simulink library "lindiPlane_lib"  (R2023b)
settings: Solver=VariableStepAuto  StartTime=0.0  StopTime=10.0  RelTol=1e-3
undefined symbols (not defined in the file or in its folder): DiscIntNeverNeededParam, lindi, lindi_notune
libraries: filters_lib x28, $bdroot x20, simulink x12, ca_lib x2, axes_transformation_lib x1, unit_conversions_lib x1, wpnav_lib x1
(part 1 of 2)
settings Model: Creator=Ybeyer  LastModifiedBy=yannic
settings SolverCC: AlgebraicLoopSolver=TrustRegion
settings DataIOCC: ReturnWorkspaceOutputs=off
settings DebuggingCC: UnconnectedInputMsg=warning  UnconnectedOutputMsg=warning  UnconnectedLineMsg=warning  ArithmeticOperatorsInVariantConditions=warning
settings ModelReferenceCC: EnableRefExpFcnMdlSchedulingChecks=on
settings SFSimCC: SimUseLocalCustomCode=off  CustomCodeUndefinedFunction=UseInterfaceOnly
settings RTWCC: RTWUseLocalCustomCode=off
settings CodeAppCC: StateflowObjectComments=on

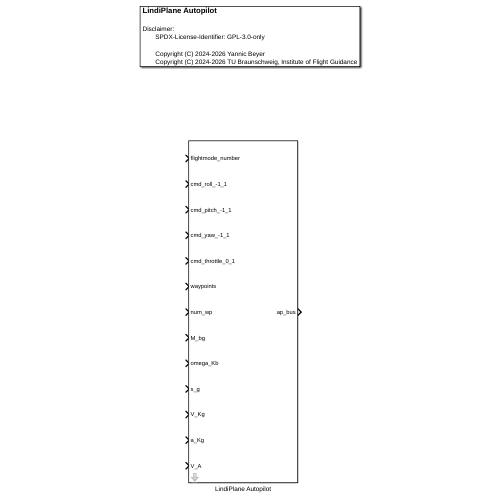
[thumbnail: Simulink's stored preview of the top-level diagram]
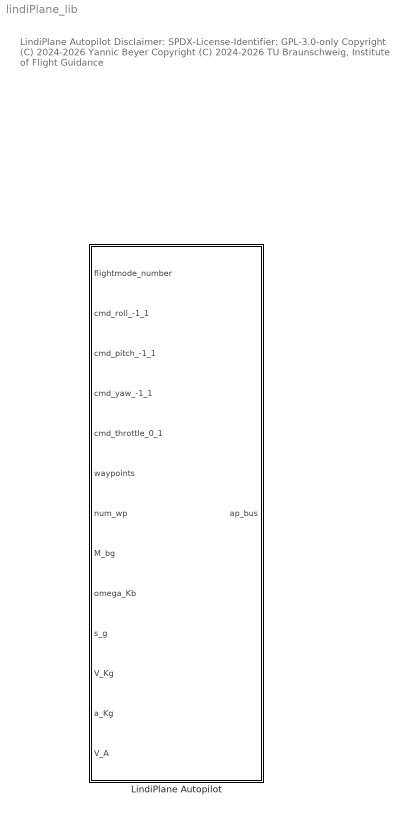
== system lindiPlane_lib ==
  note: LindiPlane Autopilot
      |
      | Disclaimer:
      | SPDX-License-Identifier: GPL-3.0-only
      |
      | Copyright (C) 2024-2026 Yannic Beyer
      | Copyright (C) 2024-2026 TU Braunschweig, Institute of Flight Guidance
  LindiPlane Autopilot : Subsystem  mask{ap=lindi, ap_notune=lindi_notune, is_enable_checked=off, states_when_enabling=reset, is_cmd_wrbm_n=off}
      mask prompts: ap "LindiPlane parameters struct, see lindiPlaneAutoCreate"; ap_notune "LindiPlane non-tunable parameters struct"; is_enable_checked "Activate "Enabled Subsystem""; states_when_enabling "States when enabling:"; is_cmd_wrbm_n "Enable WRBM load factor command"
      mask init:
      | % blockInitToggleEnable(is_enable_checked,states_when_enabling);
      | cntrlBlockInit(is_enable_checked,states_when_enabling);
      | blockInitToggleInport('cmd_WRBM_n', is_cmd_wrbm_n);
      mask Help: web('https://github.com/iff-gsc/LADAC/blob/main/control/autopilots/LindiPlane/README.md','-browser')
      mask TypeOptions states_when_enabling: held | reset
      mask DialogControl DescGroupVar Prompt: LindiPlane Autopilot
      mask DialogControl DescTextVar Prompt: The documentation of this block can be found here
      mask DialogControl Control2 Prompt: README
      mask DialogControl Control2 Callback: web('https://github.com/iff-gsc/LADAC/blob/main/control/autopilots/LindiPlane/README.md','-browser')

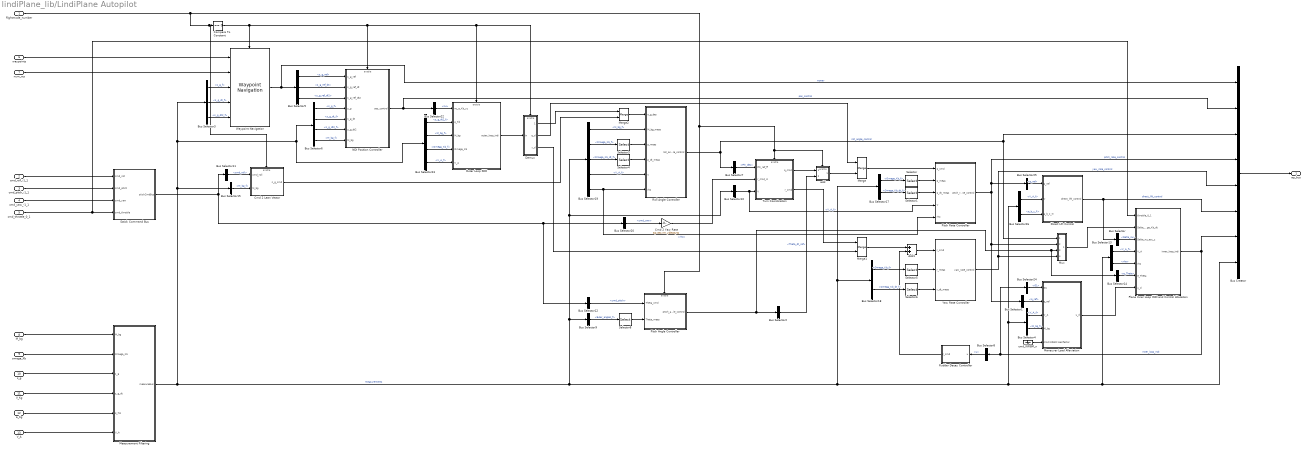
== system lindiPlane_lib/LindiPlane Autopilot ==
  flightmode_number : Inport
  cmd_roll_-1_1 : Inport  Port=2
  cmd_pitch_-1_1 : Inport  Port=3
  cmd_yaw_-1_1 : Inport  Port=4
  cmd_throttle_0_1 : Inport  Port=5
  waypoints : Inport  Port=6
  num_wp : Inport  Port=7
  M_bg : Inport  Port=8
  omega_Kb : Inport  Port=9
  s_g : Inport  Port=10
  V_Kg : Inport  Port=11
  a_Kg : Inport  Port=12
  V_A : Inport  Port=13
  Add1 : Sum
  Bus Creator : BusCreator  Inputs=8
  Bus Selector : BusSelector  OutputSignals=Delta_nu
  Bus Selector1 : BusSelector  OutputSignals=reference.q_ref
  Bus Selector10 : BusSelector  OutputSignals=V_A_f
  Bus Selector11 : BusSelector  OutputSignals=cmd_roll
  Bus Selector12 : BusSelector  OutputSignals=cmd_pitch
  Bus Selector13 : BusSelector  OutputSignals=V_A_f,rho
  Bus Selector14 : BusSelector  OutputSignals=e_Theta
  Bus Selector15 : BusSelector  OutputSignals=M_bg_f
  Bus Selector17 : BusSelector  OutputSignals=Omega_Kb_f,Omega_Kb_dt_f
  Bus Selector18 : BusSelector  OutputSignals=Omega_Kb_f,Omega_Kb_dt_f
  Bus Selector19 : BusSelector  OutputSignals=M_bg_f,Omega_Kb_f,Omega_Kb_dt_f,V_A_f,rho
  Bus Selector2 : BusSelector  OutputSignals=Theta_dt_ref
  Bus Selector20 : BusSelector  OutputSignals=cmd_yaw
  Bus Selector22 : BusSelector  OutputSignals=pseudo_control.nu
  Bus Selector23 : BusSelector  OutputSignals=s_g_dt2_f,M_bg_f,Omega_Kb_f,V_A_f
  Bus Selector24 : BusSelector  OutputSignals=G1
  Bus Selector25 : BusSelector  OutputSignals=reference.q_ref
  Bus Selector26 : BusSelector  OutputSignals=V_A_f,a_b_z_F
  Bus Selector3 : BusSelector  OutputSignals=s_g_f,s_g_dt_f,s_g_dt2_f
  Bus Selector4 : BusSelector  OutputSignals=V_A_f,M_bg_f
  Bus Selector5 : BusSelector  OutputSignals=ref_smooth.s_g_ref,ref_smooth.s_g_ref_dt,ref_smooth.s_g_ref_dt2
  Bus Selector6 : BusSelector  OutputSignals=s_g_f,s_g_dt_f,s_g_dt2_f,M_bg_f
  Bus Selector7 : BusSelector  OutputSignals=reference.Phi_des
  Bus Selector8 : BusSelector  OutputSignals=u
  Bus Selector9 : BusSelector  OutputSignals=Euler_angles_f
  Cmd 2 Lean Vector : Subsystem
  Cmd 2 Yaw Rate : Gain  Gain=ap.atc.rm.ydecaytc
  Compare To Constant : simulink/Logic and Bit Operations/Compare To Constant  relop===  const=0  OutDataTypeStr=boolean
  Demux : Subsystem
  Direct Lift Control : Subsystem
  Maneuver Load Alleviation : Subsystem
  Measurement Filtering : Subsystem
  Merge : Merge
  Merge1 : Merge
  Merge2 : Merge
  Mux : Subsystem
  NDI Position Controller : Subsystem
  Outer Loop INDI : Subsystem
  Pitch Angle Controller : Subsystem
  Pitch Rate Controller : Subsystem
  Plane Inner Loop INDI and Control Allocation : Subsystem
  Roll Angle Controller : Subsystem
  Rudder Decay Controller : Subsystem
  Selector : Selector  InputPortWidth=3  IndexOptions=Index vector (dialog)  Indices=2  OutputSizes=1
  Selector1 : Selector  InputPortWidth=3  IndexOptions=Index vector (dialog)  Indices=2  OutputSizes=1
  Selector3 : Selector  InputPortWidth=3  IndexOptions=Index vector (dialog)  Indices=1  OutputSizes=1
  Selector4 : Selector  InputPortWidth=3  IndexOptions=Index vector (dialog)  Indices=1  OutputSizes=1
  Selector5 : Selector  InputPortWidth=3  IndexOptions=Index vector (dialog)  Indices=3  OutputSizes=1
  Selector6 : Selector  InputPortWidth=3  IndexOptions=Index vector (dialog)  Indices=3  OutputSizes=1
  Selector8 : Selector  InputPortWidth=3  IndexOptions=Index vector (dialog)  Indices=2  OutputSizes=1
  Sstick Command Bus : Subsystem
  Turn Coordination : Subsystem
  Waypoint Navigation : wpnav_lib/Waypoint Navigation  wpnav=ap.wpnav  T_inner_loop=2/ap.atc.rm.rfreq + 2/(ap.servo.boost*ap.servo.omega) + 2/ap.sflt.omega  is_enable_checked=on  states_when_enabling=held  mask_expr_handling_config=passthrough (tunable)
      settings: SourceProductName=LADAC
  Yaw Rate Controller : Subsystem
  add : Subsystem
  cmd_WRBM_n : Ground
  ap_bus : Outport  VectorParamsAs1DForOutWhenUnconnected=off
  wires:
  Bus Selector15/1 -> Cmd 2 Lean Vector/2(M_bg)  "<M_bg_f>"
  cmd_WRBM_n/1 -> Maneuver Load Alleviation/5(cmd WRBM load factor)
  Bus Selector5/3 -> NDI Position Controller/3(s_g_ref_dt2)  "<s_g_ref_dt2>"
  Bus Selector5/2 -> NDI Position Controller/2(s_g_ref_dt)  "<s_g_ref_dt>"
  Bus Selector5/1 -> NDI Position Controller/1(s_g_ref)  "<s_g_ref>"
  Bus Selector14/1 -> Plane Inner Loop INDI and Control Allocation/6(e_Theta)  "<e_Theta>"
  Mux/1(Om) -> Plane Inner Loop INDI and Control Allocation/2(Delta_nu_Omega_Kb_dt)
  Bus Selector/1 -> Plane Inner Loop INDI and Control Allocation/3(Delta_nu_acc_z)  "<Delta_nu>"
  Direct Lift Control/1(direct_lift_control) -> Bus Creator/6, Bus Selector/1  "direct_lift_control"
  Bus Selector26/2 -> Direct Lift Control/3(a_b_z_N)  "<a_b_z_F>"
  Bus Selector26/1 -> Direct Lift Control/2(V)  "<V_A_f>"
  Bus Selector25/1 -> Direct Lift Control/1(q_ref)  "<q_ref>"
  waypoints/1 -> Waypoint Navigation/1
  Bus Selector19/5 -> Roll Angle Controller/6(rho), Pitch Rate Controller/5(rho)  "<rho>"
  Bus Selector19/4 -> Roll Angle Controller/5(V)  "<V_A_f>"
  Bus Selector13/2 -> Plane Inner Loop INDI and Control Allocation/5(rho)  "<rho>"
  num_wp/1 -> Waypoint Navigation/2
  NDI Position Controller/1(pos_control) -> Bus Creator/2, Bus Selector22/1  "pos_control"
  Bus Creator/1 -> ap_bus/1
  M_bg/1 -> Measurement Filtering/1(M_bg)
  omega_Kb/1 -> Measurement Filtering/2(Omega_Kb)
  s_g/1 -> Measurement Filtering/3(s_g)
  V_Kg/1 -> Measurement Filtering/4(s_g_dt)
  a_Kg/1 -> Measurement Filtering/5(a_Kg)
  V_A/1 -> Measurement Filtering/6(V_A)
  Bus Selector12/1 -> Pitch Angle Controller/1(Theta_cmd)  "<cmd_pitch>"
  Bus Selector6/2 -> NDI Position Controller/5(s_g_dt)  "<s_g_dt_f>"
  Measurement Filtering/1(measureBus) -> Bus Selector19/1, Bus Selector10/1, Bus Selector9/1, Bus Selector17/1, Bus Selector18/1, Bus Creator/8, Bus Selector13/1, Bus Selector4/1, Bus Selector26/1, Bus Selector23/1, Bus Selector6/1, Bus Selector3/1, Bus Selector15/1  "measurements"
  Bus Selector8/1 -> Rudder Decay Controller/1(u)  "<u>"
  Yaw Rate Controller/1(yaw_rate_control) -> Mux/4(yaw), Bus Creator/5  "yaw_rate_control"
  cmd_yaw_-1_1/1 -> Sstick Command Bus/3(cmd_yaw)
  Bus Selector13/1 -> Plane Inner Loop INDI and Control Allocation/4(V_A)  "<V_A_f>"
  flightmode_number/1 -> Cmd 2 Lean Vector/Enable, Compare To Constant/1, add/Enable, Turn Coordination/Enable, Pitch Angle Controller/Enable
  Bus Selector18/2 -> Selector6/1  "<Omega_Kb_dt_f>"
  Selector4/1 -> Roll Angle Controller/4(p_dt_meas)
  Cmd 2 Lean Vector/1(n_g_cmd) -> Merge2/2
  Bus Selector3/2 -> Waypoint Navigation/4  "<s_g_dt_f>"
  Bus Selector17/1 -> Selector/1  "<Omega_Kb_f>"
  Selector6/1 -> Yaw Rate Controller/3(r_dt_meas)
  Selector5/1 -> Yaw Rate Controller/2(r_meas)
  Roll Angle Controller/1(roll_angle_control) -> Bus Creator/3, Mux/1(rll), Bus Selector7/1  "roll_angle_control"
  Merge1/1 -> Add1/1
  Selector8/1 -> Pitch Angle Controller/2(Theta_meas)
  cmd_throttle_0_1/1 -> Plane Inner Loop INDI and Control Allocation/1(throttle_0_1), Sstick Command Bus/4(cmd_throttle)
  Pitch Rate Controller/1(pitch_rate_control) -> Mux/2(ptch), Bus Selector1/1, Bus Selector25/1, Bus Creator/4  "pitch_rate_control"
  Bus Selector6/3 -> NDI Position Controller/6(s_g_dt2)  "<s_g_dt2_f>"
  Turn Coordination/2(r_cmd) -> Merge1/1
  Selector3/1 -> Roll Angle Controller/3(p_meas)
  Waypoint Navigation/1 -> Bus Selector5/1, Bus Creator/1  "wpnav"
  Bus Selector10/1 -> Turn Coordination/3(V), Pitch Rate Controller/4(V)  "<V_A_f>"
  Selector1/1 -> Pitch Rate Controller/3(q_dt_meas)
  cmd_pitch_-1_1/1 -> Sstick Command Bus/2(cmd_pitch)
  Selector/1 -> Pitch Rate Controller/2(q_meas)
  Bus Selector19/2 -> Selector3/1  "<Omega_Kb_f>"
  Compare To Constant/1 -> Waypoint Navigation/Enable, Demux/Enable, Outer Loop INDI/Enable, NDI Position Controller/Enable
  Cmd 2 Yaw Rate/1 -> Turn Coordination/2(r_cmd_in)
  Bus Selector3/1 -> Waypoint Navigation/3  "<s_g_f>"
  Sstick Command Bus/1(stickCmdBus) -> Bus Selector11/1, Bus Selector20/1, Bus Selector12/1
  Bus Selector9/1 -> Selector8/1  "<Euler_angles_f>"
  Rudder Decay Controller/1(r_cmd) -> Add1/2
  Bus Selector19/3 -> Selector4/1  "<Omega_Kb_dt_f>"
  Bus Selector17/2 -> Selector1/1  "<Omega_Kb_dt_f>"
  Bus Selector11/1 -> Cmd 2 Lean Vector/1(cmd_roll)  "<cmd_roll>"
  Bus Selector2/1 -> add/2(In2)  "<Theta_dt_ref>"
  cmd_roll_-1_1/1 -> Sstick Command Bus/1(cmd_roll)
  Bus Selector19/1 -> Roll Angle Controller/2(M_bg_meas)  "<M_bg_f>"
  Bus Selector6/1 -> NDI Position Controller/4(s_g)  "<s_g_f>"
  Plane Inner Loop INDI and Control Allocation/1(inner_loop_indi) -> Bus Creator/7, Bus Selector8/1, Bus Selector24/1  "inner_loop_indi"
  Bus Selector6/4 -> NDI Position Controller/7(M_bg)  "<M_bg_f>"
  Bus Selector18/1 -> Selector5/1  "<Omega_Kb_f>"
  Add1/1 -> Yaw Rate Controller/1(r_cmd)
  Merge2/1 -> Roll Angle Controller/1(n_g_des)
  Bus Selector20/1 -> Cmd 2 Yaw Rate/1  "<cmd_yaw>"
  Bus Selector3/3 -> Waypoint Navigation/5  "<s_g_dt2_f>"
  Merge/1 -> Pitch Rate Controller/1(q_cmd)
  Turn Coordination/1(q_cmd) -> add/1(In1)
  add/1(Out1) -> Merge/2
  Pitch Angle Controller/1(pitch_angle_control) -> Bus Selector2/1, Mux/3(ptch2), Bus Selector14/1
  Outer Loop INDI/1(outer_loop_indi) -> Demux/1(In)
  Demux/2(q_d) -> Merge/1
  Demux/3(r_d) -> Merge1/2
  Demux/1(n_g_d) -> Merge2/1
  Bus Selector7/1 -> Turn Coordination/1(Phi_ref_ff)  "<Phi_des>"
  Bus Selector22/1 -> Outer Loop INDI/1(nu_a_Kb_yz)  "<nu>"
  Bus Selector23/4 -> Outer Loop INDI/5(V_A)  "<V_A_f>"
  Bus Selector23/3 -> Outer Loop INDI/4(Omega_Kb)  "<Omega_Kb_f>"
  Bus Selector23/2 -> Outer Loop INDI/3(M_bg)  "<M_bg_f>"
  Bus Selector23/1 -> Outer Loop INDI/2(a_Kb)  "<s_g_dt2_f>"
  Bus Selector1/1 -> Maneuver Load Alleviation/2(q_ref)  "<q_ref>"
  Bus Selector4/1 -> Maneuver Load Alleviation/3(V_A)  "<V_A_f>"
  Bus Selector4/2 -> Maneuver Load Alleviation/4(M_bg)  "<M_bg_f>"
  Bus Selector24/1 -> Maneuver Load Alleviation/1(G1)  "<G1>"
  Maneuver Load Alleviation/1(u_d) -> Plane Inner Loop INDI and Control Allocation/7(u_d)

== system lindiPlane_lib/LindiPlane Autopilot/Cmd 2 Lean Vector ==
  cmd_roll : Inport
  M_bg : Inport  Port=2
  Enable : EnablePort
  Cmd Roll 2 n_g_cmd : MATLAB Function  TreatAsAtomicUnit=on
  Gain : Gain  Gain=ap.atc.rm.rangmax*pi/180
  n_g_cmd : Outport  VectorParamsAs1DForOutWhenUnconnected=off
  wires:
  M_bg/1 -> Cmd Roll 2 n_g_cmd/2(M_bg)
  Cmd Roll 2 n_g_cmd/1(n_g_cmd) -> n_g_cmd/1
  Gain/1 -> Cmd Roll 2 n_g_cmd/1(Phi_cmd)
  cmd_roll/1 -> Gain/1

== system lindiPlane_lib/LindiPlane Autopilot/Demux ==
  In : Inport
  Enable : EnablePort
  Bus Selector24 : BusSelector  OutputSignals=n_g_des,q_des,r_des
  n_g_d : Outport  VectorParamsAs1DForOutWhenUnconnected=off
  q_d : Outport  Port=2  VectorParamsAs1DForOutWhenUnconnected=off
  r_d : Outport  Port=3  VectorParamsAs1DForOutWhenUnconnected=off
  wires:
  Bus Selector24/1 -> n_g_d/1  "<n_g_des>"
  In/1 -> Bus Selector24/1
  Bus Selector24/2 -> q_d/1  "<q_des>"
  Bus Selector24/3 -> r_d/1  "<r_des>"

== system lindiPlane_lib/LindiPlane Autopilot/Direct Lift Control ==
  q_ref : Inport
  V : Inport  Port=2
  a_b_z_N : Inport  Port=3
  Acc Filter : $bdroot/LindiPlane Autopilot/Measurement Filtering/Acc Filter  SystemSampleTime=-1  VariantActivationTime=update diagram  AllowFlexibleInterface=on  Latency=0  AutoFrameSizeCalculation=off
  Add : Sum  Inputs=|+-
  Bus Creator : BusCreator  Inputs=4
  Gain1 : Gain  Gain=-1
  Product : Product
  Scope : Scope  NumInputPorts=3
  direct_lift_control : Outport  VectorParamsAs1DForOutWhenUnconnected=off
  wires:
  Acc Filter/1 -> Scope/2, Bus Creator/2  "nu_f"
  Gain1/1 -> Scope/1, Bus Creator/1, Acc Filter/1, Add/1  "nu"
  a_b_z_N/1 -> Scope/3, Bus Creator/4, Add/2  "nu_meas"
  Add/1 -> Bus Creator/3  "Delta_nu"
  V/1 -> Product/2
  Product/1 -> Gain1/1
  Bus Creator/1 -> direct_lift_control/1
  q_ref/1 -> Product/1

== system lindiPlane_lib/LindiPlane Autopilot/Maneuver Load Alleviation ==
  G1 : Inport
  q_ref : Inport  Port=2
  V_A : Inport  Port=3
  M_bg : Inport  Port=4
  cmd WRBM load factor : Inport  Port=5
  Compare To Constant : simulink/Logic and Bit Operations/Compare To Constant  relop===  const=0  OutDataTypeStr=boolean
  Constant : Constant  Value=ap.mla.use
  Logical Operator : Logic  Operator=NOT  AllPortsSameDT=off  OutDataTypeStr=boolean
  Maneuver Load Alleviation : Subsystem  mask{ca_main=ap.ca, ca_mla=ap.mla.ca}
      mask prompts: ca_main "Control allocation struct (main)"; ca_mla "Control allocation struct (MLA)"
      mask DialogControl DescGroupVar Prompt: Maneuver Load Alleviation (MLA)
  Merge : Merge
  Subsystem : Subsystem
  u_d : Outport  VectorParamsAs1DForOutWhenUnconnected=off
  wires:
  cmd WRBM load factor/1 -> Maneuver Load Alleviation/5(cmd WRBM load factor)
  M_bg/1 -> Maneuver Load Alleviation/4(M_bg)
  G1/1 -> Maneuver Load Alleviation/1(G1)
  q_ref/1 -> Maneuver Load Alleviation/3(q_ref)
  V_A/1 -> Maneuver Load Alleviation/2(V_A)
  Compare To Constant/1 -> Logical Operator/1, Subsystem/Enable
  Subsystem/1(u_d) -> Merge/1
  Constant/1 -> Compare To Constant/1
  Maneuver Load Alleviation/1(u_d) -> Merge/2
  Merge/1 -> u_d/1
  Logical Operator/1 -> Maneuver Load Alleviation/Enable

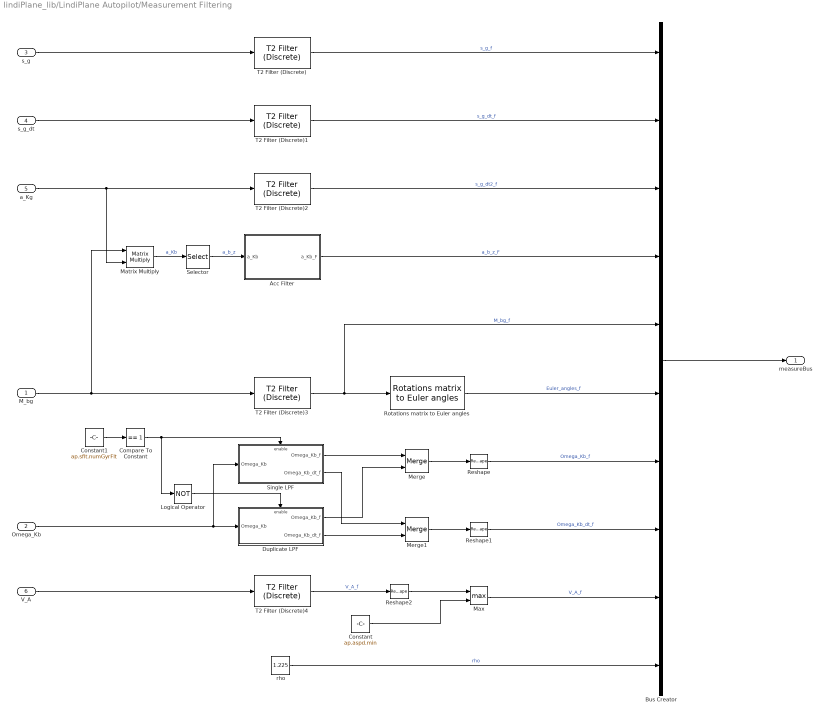
== system lindiPlane_lib/LindiPlane Autopilot/Measurement Filtering ==
  M_bg : Inport
  Omega_Kb : Inport  Port=2
  s_g : Inport  Port=3
  s_g_dt : Inport  Port=4
  a_Kg : Inport  Port=5
  V_A : Inport  Port=6
  Acc Filter : Subsystem
  Bus Creator : BusCreator  Inputs=10
  Compare To Constant : simulink/Logic and Bit Operations/Compare To Constant  relop===  const=1  OutDataTypeStr=boolean
  Constant : Constant  Value=ap.aspd.min
  Constant1 : Constant  Value=ap.sflt.numGyrFlt
  Duplicate LPF : Subsystem
  Logical Operator : Logic  Operator=NOT  AllPortsSameDT=off  OutDataTypeStr=boolean
  Matrix Multiply : Product  Multiplication=Matrix(*)
  Max : MinMax  Function=max  Inputs=2
  Merge : Merge
  Merge1 : Merge
  Reshape : Reshape  OutputDimensionality=Column vector (2-D)
  Reshape1 : Reshape  OutputDimensionality=Column vector (2-D)
  Reshape2 : Reshape
  Rotations matrix to Euler angles : axes_transformation_lib/Rotations matrix to Euler angles  SystemSampleTime=-1  VariantActivationTime=update diagram  AllowFlexibleInterface=on  Latency=0  AutoFrameSizeCalculation=off
      settings: SourceProductName=LADAC
  Selector : Selector  InputPortWidth=3  IndexOptions=Index vector (dialog)  Indices=3  OutputSizes=1
  Single LPF : Subsystem
  T2 Filter (Discrete){,1..3} (4 alike) : filters_lib/T2 Filter (Discrete)  omega_0=ap.sflt.omega  d=ap.sflt.d  Ts=ap_notune.ts  is_vel=false  is_acc=false  SimulateUsing=Code generation
      settings: SourceProductName=LADAC
  T2 Filter (Discrete)4 : filters_lib/T2 Filter (Discrete)  omega_0=2/ap.aspd.flttc  d=1  Ts=ap_notune.ts  is_vel=false  is_acc=false  SimulateUsing=Code generation
      settings: SourceProductName=LADAC
  rho : Constant  Value=1.225
  measureBus : Outport  VectorParamsAs1DForOutWhenUnconnected=off
  wires:
  Reshape2/1 -> Max/1
  Acc Filter/1(a_Kb_F) -> Bus Creator/4  "a_b_z_F"
  Selector/1 -> Acc Filter/1(a_Kb)  "a_b_z"
  Matrix Multiply/1 -> Selector/1  "a_Kb"
  M_bg/1 -> Matrix Multiply/1, T2 Filter (Discrete)3/1
  a_Kg/1 -> Matrix Multiply/2, T2 Filter (Discrete)2/1
  Logical Operator/1 -> Duplicate LPF/Enable
  Compare To Constant/1 -> Single LPF/Enable, Logical Operator/1
  Duplicate LPF/2(Omega_Kb_dt_f) -> Merge1/2
  Single LPF/2(Omega_Kb_dt_f) -> Merge1/1
  Duplicate LPF/1(Omega_Kb_f) -> Merge/2
  Single LPF/1(Omega_Kb_f) -> Merge/1
  Omega_Kb/1 -> Duplicate LPF/1(Omega_Kb), Single LPF/1(Omega_Kb)
  Constant1/1 -> Compare To Constant/1
  Reshape1/1 -> Bus Creator/8  "Omega_Kb_dt_f"
  Reshape/1 -> Bus Creator/7  "Omega_Kb_f"
  Merge/1 -> Reshape/1
  rho/1 -> Bus Creator/10  "rho"
  Constant/1 -> Max/2
  T2 Filter (Discrete)4/1 -> Reshape2/1  "V_A_f"
  Max/1 -> Bus Creator/9  "V_A_f"
  T2 Filter (Discrete)1/1 -> Bus Creator/2  "s_g_dt_f"
  T2 Filter (Discrete)/1 -> Bus Creator/1  "s_g_f"
  Bus Creator/1 -> measureBus/1
  T2 Filter (Discrete)2/1 -> Bus Creator/3  "s_g_dt2_f"
  Merge1/1 -> Reshape1/1
  V_A/1 -> T2 Filter (Discrete)4/1
  s_g/1 -> T2 Filter (Discrete)/1
  Rotations matrix to Euler angles/1 -> Bus Creator/6  "Euler_angles_f"
  T2 Filter (Discrete)3/1 -> Rotations matrix to Euler angles/1, Bus Creator/5  "M_bg_f"
  s_g_dt/1 -> T2 Filter (Discrete)1/1

== system lindiPlane_lib/LindiPlane Autopilot/Mux ==
  rll : Inport
  ptch : Inport  Port=2
  ptch2 : Inport  Port=3
  yaw : Inport  Port=4
  Add : Sum
  Bus Selector14 : BusSelector  OutputSignals=pseudo_control.Delta_nu
  Bus Selector15 : BusSelector  OutputSignals=pseudo_control.Delta_nu
  Bus Selector16 : BusSelector  OutputSignals=pseudo_control.Delta_nu
  Bus Selector21 : BusSelector  OutputSignals=nu_q_dt_ptchcntrl
  Mux2 : Mux  Inputs=3
  Om : Outport  VectorParamsAs1DForOutWhenUnconnected=off
  wires:
  ptch/1 -> Bus Selector15/1
  Bus Selector21/1 -> Add/2  "<nu_q_dt_ptchcntrl>"
  ptch2/1 -> Bus Selector21/1
  rll/1 -> Bus Selector14/1
  Bus Selector14/1 -> Mux2/1  "<Delta_nu>"
  yaw/1 -> Bus Selector16/1
  Mux2/1 -> Om/1
  Bus Selector16/1 -> Mux2/3  "<Delta_nu>"
  Add/1 -> Mux2/2
  Bus Selector15/1 -> Add/1  "<Delta_nu>"

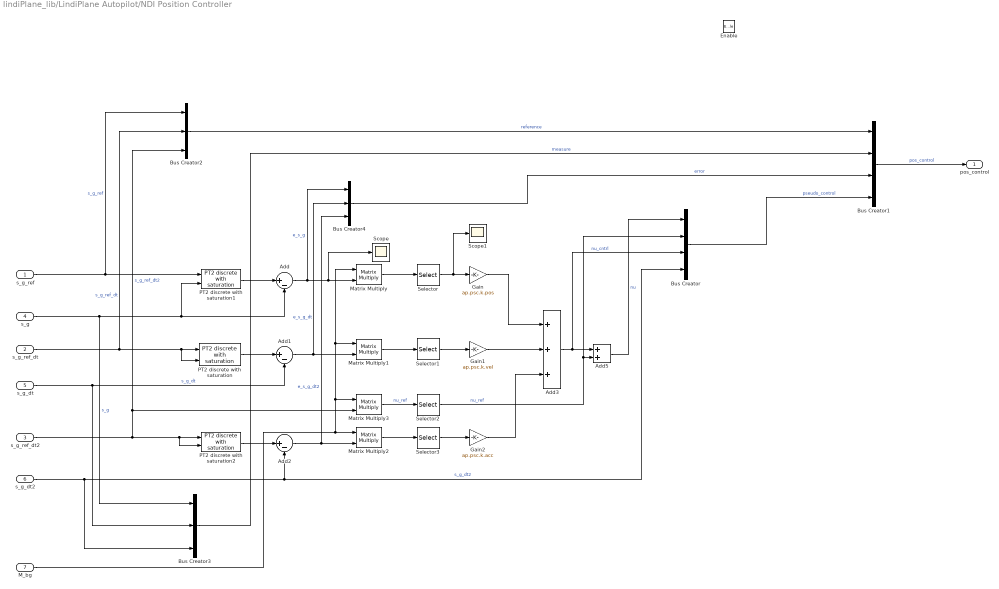
== system lindiPlane_lib/LindiPlane Autopilot/NDI Position Controller ==
  s_g_ref : Inport
  s_g_ref_dt : Inport  Port=2
  s_g_ref_dt2 : Inport  Port=3
  s_g : Inport  Port=4
  s_g_dt : Inport  Port=5
  s_g_dt2 : Inport  Port=6
  M_bg : Inport  Port=7
  Enable : EnablePort  StatesWhenEnabling=reset
  Add : Sum  Inputs=|+-
  Add1 : Sum  Inputs=|+-
  Add2 : Sum  Inputs=|+-
  Add3 : Sum  Inputs=+++
  Add5 : Sum
  Bus Creator : BusCreator  Inputs=4
  Bus Creator1 : BusCreator  Inputs=4
  Bus Creator2 : BusCreator  Inputs=3
  Bus Creator3 : BusCreator  Inputs=3
  Bus Creator4 : BusCreator  Inputs=3
  Gain : Gain  Gain=ap.psc.k.pos
  Gain1 : Gain  Gain=ap.psc.k.vel
  Gain2 : Gain  Gain=ap.psc.k.acc
  Matrix Multiply{,1..3} (4 alike) : Product  Multiplication=Matrix(*)
  PT2 discrete with saturation : filters_lib/PT2 discrete with saturation  param_src=internal  omega=2/(2/ap.atc.rm.rfreq+2/(ap.servo.omega*ap.servo.boost)+2/ap.sflt.omega)  d=1  x_max=inf  x_min=-inf  x_dt_max=inf  x_dt_min=-inf  x_dt2_max=inf  x_dt2_min=-inf  y_0_src=external  x_init=0  y_dt_0_src=internal  x_dt_init=0  is_y_dt_checked=off  is_y_dt2_checked=off  is_external_reset_checked=off  mask_expr_handling_config=default
      settings: SourceProductName=LADAC
  PT2 discrete with saturation1 : filters_lib/PT2 discrete with saturation  param_src=internal  omega=2/(2/ap.atc.rm.rfreq+2/(ap.servo.omega*ap.servo.boost)+2/ap.sflt.omega)  d=1  x_max=inf  x_min=-inf  x_dt_max=inf  x_dt_min=-inf  x_dt2_max=inf  x_dt2_min=-inf  y_0_src=external  x_init=0  y_dt_0_src=internal  x_dt_init=0  is_y_dt_checked=off  is_y_dt2_checked=off  is_external_reset_checked=off  mask_expr_handling_config=default
      settings: SourceProductName=LADAC
  PT2 discrete with saturation2 : filters_lib/PT2 discrete with saturation  param_src=internal  omega=2/(2/ap.atc.rm.rfreq+2/(ap.servo.omega*ap.servo.boost)+2/ap.sflt.omega)  d=1  x_max=inf  x_min=-inf  x_dt_max=inf  x_dt_min=-inf  x_dt2_max=inf  x_dt2_min=-inf  y_0_src=external  x_init=0  y_dt_0_src=internal  x_dt_init=0  is_y_dt_checked=off  is_y_dt2_checked=off  is_external_reset_checked=off  mask_expr_handling_config=default
      settings: SourceProductName=LADAC
  Scope : Scope
  Scope1 : Scope
  Selector{,1..3} (4 alike) : Selector  InputPortWidth=3  IndexOptions=Index vector (dialog)  Indices=[2,3]  OutputSizes=1
  pos_control : Outport  VectorParamsAs1DForOutWhenUnconnected=off
  wires:
  Bus Creator4/1 -> Bus Creator1/3  "error"
  Bus Creator1/1 -> pos_control/1  "pos_control"
  Selector3/1 -> Gain2/1
  Selector2/1 -> Add5/2, Bus Creator/2  "nu_ref"
  Selector1/1 -> Gain1/1
  Selector/1 -> Gain/1, Scope1/1
  Bus Creator3/1 -> Bus Creator1/2  "measure"
  Bus Creator2/1 -> Bus Creator1/1  "reference"
  Add5/1 -> Bus Creator/1  "nu"
  Bus Creator/1 -> Bus Creator1/4  "pseudo_control"
  Matrix Multiply3/1 -> Selector2/1  "nu_ref"
  s_g_ref_dt2/1 -> Bus Creator2/3, Matrix Multiply3/2, PT2 discrete with saturation2/1, PT2 discrete with saturation2/2  "s_g_ref_dt2"
  PT2 discrete with saturation2/1 -> Add2/1
  PT2 discrete with saturation1/1 -> Add/1
  PT2 discrete with saturation/1 -> Add1/1
  M_bg/1 -> Matrix Multiply1/1, Matrix Multiply/1, Matrix Multiply3/1, Matrix Multiply2/1
  s_g_ref/1 -> Bus Creator2/1, PT2 discrete with saturation1/1  "s_g_ref"
  Add/1 -> Bus Creator4/1, Scope/1, Matrix Multiply/2  "e_s_g"
  s_g_ref_dt/1 -> Bus Creator2/2, PT2 discrete with saturation/1, PT2 discrete with saturation/2  "s_g_ref_dt"
  Add1/1 -> Bus Creator4/2, Matrix Multiply1/2  "e_s_g_dt"
  s_g_dt2/1 -> Add2/2, Bus Creator/4, Bus Creator3/3  "s_g_dt2"
  s_g_dt/1 -> Add1/2, Bus Creator3/2  "s_g_dt"
  Matrix Multiply2/1 -> Selector3/1
  Gain2/1 -> Add3/3
  Gain1/1 -> Add3/2
  Matrix Multiply/1 -> Selector/1
  Add3/1 -> Add5/1, Bus Creator/3  "nu_cntrl"
  Add2/1 -> Matrix Multiply2/2, Bus Creator4/3  "e_s_g_dt2"
  Matrix Multiply1/1 -> Selector1/1
  Gain/1 -> Add3/1
  s_g/1 -> PT2 discrete with saturation1/2, Add/2, Bus Creator3/1  "s_g"

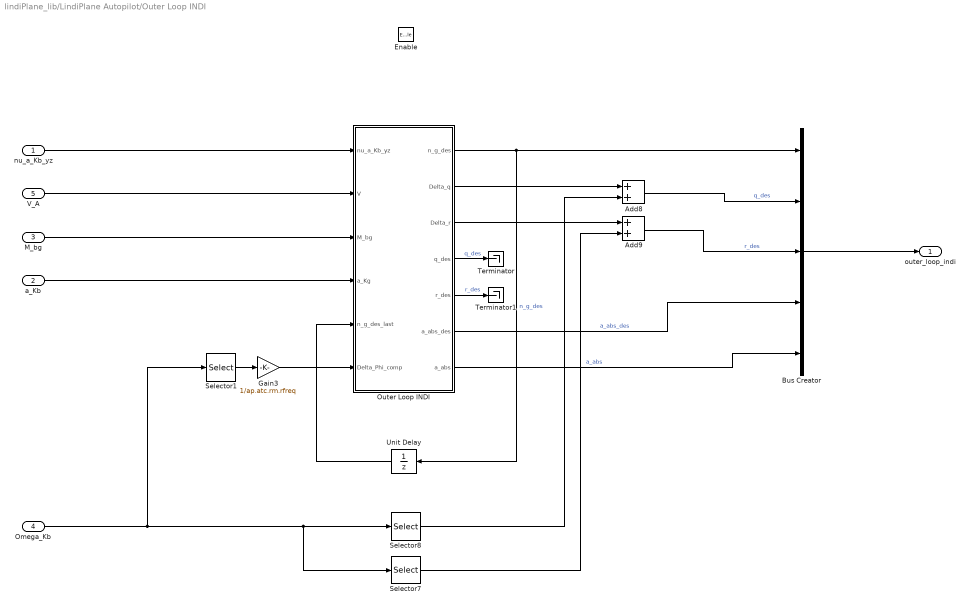
== system lindiPlane_lib/LindiPlane Autopilot/Outer Loop INDI ==
  nu_a_Kb_yz : Inport
  a_Kb : Inport  Port=2
  M_bg : Inport  Port=3
  Omega_Kb : Inport  Port=4
  V_A : Inport  Port=5
  Enable : EnablePort  StatesWhenEnabling=reset
  Add8 : Sum
  Add9 : Sum
  Bus Creator : BusCreator  Inputs=5
  Gain3 : Gain  Gain=1/ap.atc.rm.rfreq
  Outer Loop INDI : MATLAB Function  TreatAsAtomicUnit=on
  Selector1 : Selector  InputPortWidth=3  IndexOptions=Index vector (dialog)  Indices=1  OutputSizes=1
  Selector7 : Selector  InputPortWidth=3  IndexOptions=Index vector (dialog)  Indices=3  OutputSizes=1
  Selector8 : Selector  InputPortWidth=3  IndexOptions=Index vector (dialog)  Indices=2  OutputSizes=1
  Terminator : Terminator
  Terminator1 : Terminator
  Unit Delay : UnitDelay  SampleTime=-1  HasFrameUpgradeWarning=on
  outer_loop_indi : Outport  VectorParamsAs1DForOutWhenUnconnected=off
  wires:
  Outer Loop INDI/5(r_des) -> Terminator1/1  "r_des"
  Outer Loop INDI/4(q_des) -> Terminator/1  "q_des"
  Outer Loop INDI/2(Delta_q) -> Add8/1
  Gain3/1 -> Outer Loop INDI/6(Delta_Phi_comp)
  Selector1/1 -> Gain3/1
  Outer Loop INDI/1(n_g_des) -> Bus Creator/1, Unit Delay/1  "n_g_des"
  Unit Delay/1 -> Outer Loop INDI/5(n_g_des_last)
  Outer Loop INDI/6(a_abs_des) -> Bus Creator/4  "a_abs_des"
  nu_a_Kb_yz/1 -> Outer Loop INDI/1(nu_a_Kb_yz)
  Selector8/1 -> Add8/2
  Outer Loop INDI/7(a_abs) -> Bus Creator/5  "a_abs"
  Outer Loop INDI/3(Delta_r) -> Add9/1
  Add9/1 -> Bus Creator/3  "r_des"
  Omega_Kb/1 -> Selector8/1, Selector7/1, Selector1/1
  Add8/1 -> Bus Creator/2  "q_des"
  V_A/1 -> Outer Loop INDI/2(V)
  Selector7/1 -> Add9/2
  a_Kb/1 -> Outer Loop INDI/4(a_Kg)
  M_bg/1 -> Outer Loop INDI/3(M_bg)
  Bus Creator/1 -> outer_loop_indi/1

== system lindiPlane_lib/LindiPlane Autopilot/Pitch Angle Controller ==
  Theta_cmd : Inport
  Theta_meas : Inport  Port=2
  Enable : EnablePort  StatesWhenEnabling=reset
  Add3 : Sum  Inputs=|+-
  Bus Creator : BusCreator  Inputs=4
  Gain : Gain  Gain=ap.atc.k.pang
  PT1 discrete with saturations : filters_lib/PT1 discrete with saturations  param_src=internal  T=1/ap.atc.rm.pfreq  x_max=inf  x_min=-inf  x_dt_max=inf  x_dt_min=-inf  y_0_src=external  x_init=0  is_y_dt_checked=on  is_external_reset_checked=off  mask_expr_handling_config=passthrough (tunable)
      settings: SourceProductName=LADAC
  PT1 discrete with saturations1 : filters_lib/PT1 discrete with saturations  param_src=internal  T=1/ap.atc.rm.pfreq  x_max=inf  x_min=-inf  x_dt_max=inf  x_dt_min=-inf  y_0_src=external  x_init=0  is_y_dt_checked=off  is_external_reset_checked=off  mask_expr_handling_config=passthrough (tunable)
      settings: SourceProductName=LADAC
  Servo and Sensor Filter Delay : Subsystem
  Terminator : Terminator
  Terminator1 : Terminator
  cmd 2 angle : Gain  Gain=ap.atc.rm.pangmax*pi/180
  pitch_angle_control : Outport  VectorParamsAs1DForOutWhenUnconnected=off
  wires:
  Servo and Sensor Filter Delay/3(ref_dt2_f) -> Terminator1/1
  Servo and Sensor Filter Delay/2(ref_dt_f) -> Terminator/1
  Theta_cmd/1 -> cmd 2 angle/1
  PT1 discrete with saturations/1 -> PT1 discrete with saturations1/2, PT1 discrete with saturations1/1
  PT1 discrete with saturations/2 -> Bus Creator/4  "Theta_dt_ref"
  cmd 2 angle/1 -> PT1 discrete with saturations/2, PT1 discrete with saturations/1
  PT1 discrete with saturations1/1 -> Servo and Sensor Filter Delay/1(ref), Bus Creator/1  "Theta_ref"
  Servo and Sensor Filter Delay/1(ref_f) -> Add3/1
  Add3/1 -> Gain/1, Bus Creator/2  "e_Theta"
  Theta_meas/1 -> Add3/2
  Gain/1 -> Bus Creator/3  "nu_q_dt_ptchcntrl"
  Bus Creator/1 -> pitch_angle_control/1  "pitch_angle_control"

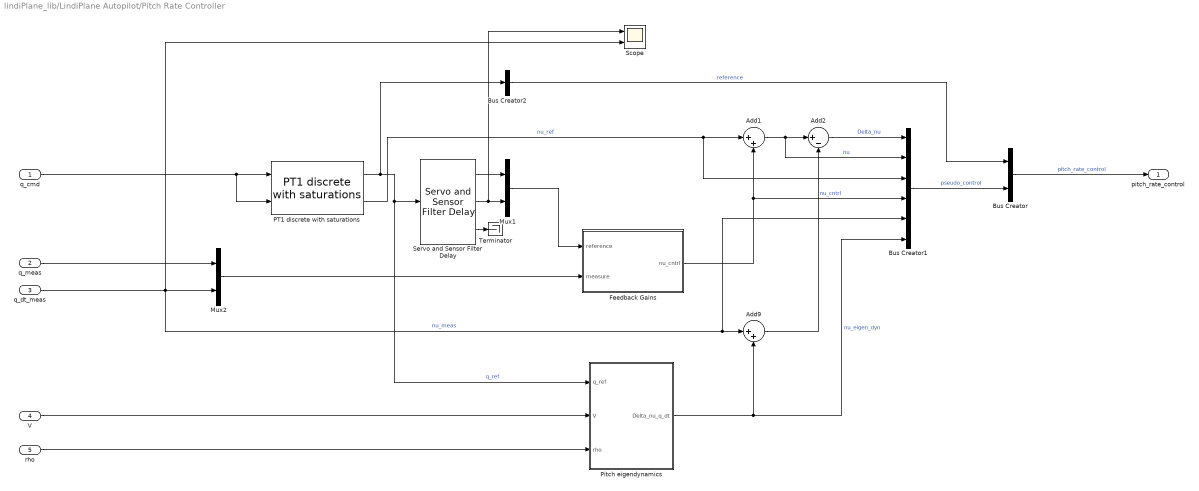
== system lindiPlane_lib/LindiPlane Autopilot/Pitch Rate Controller ==
  q_cmd : Inport
  q_meas : Inport  Port=2
  q_dt_meas : Inport  Port=3
  V : Inport  Port=4
  rho : Inport  Port=5
  Add1 : Sum  Inputs=|++
  Add2 : Sum  Inputs=|+-
  Add9 : Sum  Inputs=|++
  Bus Creator : BusCreator  Inputs=2
  Bus Creator1 : BusCreator  Inputs=6
  Bus Creator2 : BusCreator  Inputs=1
  Feedback Gains : Subsystem
  Mux1 : Mux  Inputs=2
  Mux2 : Mux  Inputs=2
  PT1 discrete with saturations : filters_lib/PT1 discrete with saturations  param_src=internal  T=1/ap.atc.rm.pfreq  x_max=inf  x_min=-inf  x_dt_max=inf  x_dt_min=-inf  y_0_src=external  x_init=0  is_y_dt_checked=on  is_external_reset_checked=off  mask_expr_handling_config=passthrough (tunable)
      settings: SourceProductName=LADAC
  Pitch eigendynamics : Subsystem
  Scope : Scope  NumInputPorts=2
  Servo and Sensor Filter Delay : $bdroot/LindiPlane Autopilot/Pitch Angle Controller/Servo and Sensor Filter Delay  SystemSampleTime=-1  VariantActivationTime=update diagram  AllowFlexibleInterface=on  Latency=0  AutoFrameSizeCalculation=off
  Terminator : Terminator
  pitch_rate_control : Outport  VectorParamsAs1DForOutWhenUnconnected=off
  wires:
  Servo and Sensor Filter Delay/3 -> Terminator/1
  Servo and Sensor Filter Delay/1 -> Mux1/1
  Servo and Sensor Filter Delay/2 -> Mux1/2, Scope/1
  PT1 discrete with saturations/2 -> Bus Creator1/3, Add1/1  "nu_ref"
  Mux1/1 -> Feedback Gains/1(reference)
  Add1/1 -> Add2/1, Bus Creator1/2  "nu"
  Bus Creator1/1 -> Bus Creator/2  "pseudo_control"
  Bus Creator/1 -> pitch_rate_control/1  "pitch_rate_control"
  Add2/1 -> Bus Creator1/1  "Delta_nu"
  q_cmd/1 -> PT1 discrete with saturations/1, PT1 discrete with saturations/2
  q_meas/1 -> Mux2/1
  q_dt_meas/1 -> Bus Creator1/5, Add9/1, Mux2/2, Scope/2  "nu_meas"
  Feedback Gains/1(nu_cntrl) -> Add1/2, Bus Creator1/4  "nu_cntrl"
  Mux2/1 -> Feedback Gains/2(measure)
  Bus Creator2/1 -> Bus Creator/1  "reference"
  Pitch eigendynamics/1(Delta_nu_q_dt) -> Bus Creator1/6, Add9/2  "nu_eigen_dyn"
  Add9/1 -> Add2/2
  rho/1 -> Pitch eigendynamics/3(rho)
  V/1 -> Pitch eigendynamics/2(V)
  PT1 discrete with saturations/1 -> Bus Creator2/1, Servo and Sensor Filter Delay/1, Pitch eigendynamics/1(q_ref)  "q_ref"

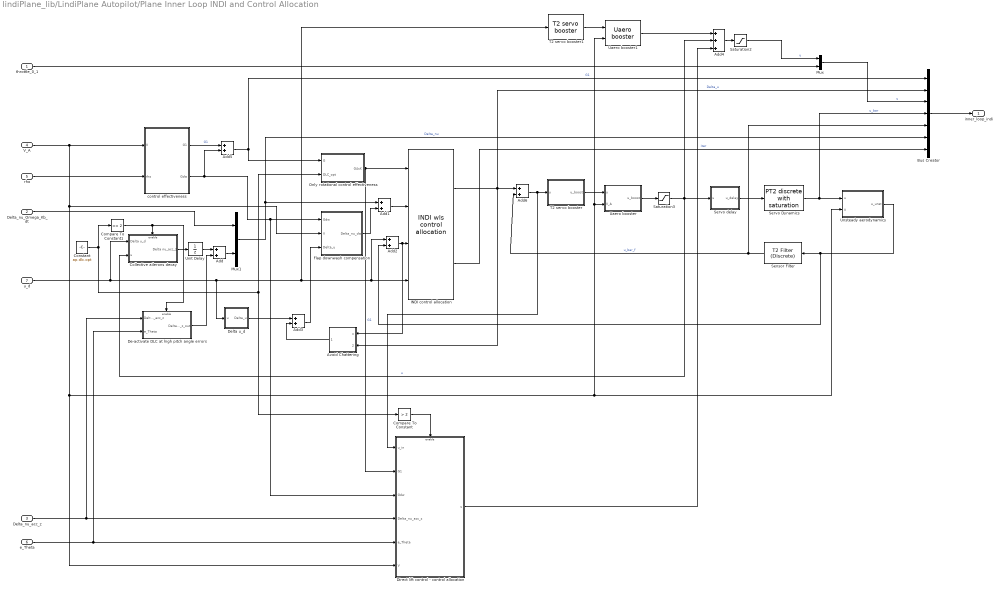
== system lindiPlane_lib/LindiPlane Autopilot/Plane Inner Loop INDI and Control Allocation ==
  throttle_0_1 : Inport
  Delta_nu_Omega_Kb_dt : Inport  Port=2
  Delta_nu_acc_z : Inport  Port=3
  V_A : Inport  Port=4
  rho : Inport  Port=5
  e_Theta : Inport  Port=6
  u_d : Inport  Port=7
  Add{,1..3,5..6} (6 alike) : Sum
  Add4 : Sum  Inputs=+++
  Avoid Chattering : Subsystem
  Bus Creator : BusCreator  Inputs=7
  Collective ailerons decay : Subsystem
  Compare To Constant : simulink/Logic and Bit Operations/Compare To Constant  relop=>  const=2  OutDataTypeStr=boolean
  Compare To Constant1 : simulink/Logic and Bit Operations/Compare To Constant  relop===  const=2  OutDataTypeStr=boolean
  Constant : Constant  Value=ap.dlc.opt
  De-activate DLC at high pitch angle errors : Subsystem
  Delta u_d : Subsystem
  Direct lift control - control allocation : Subsystem
  Flap downwash compensation : Subsystem  mask{ceb=ap.ceb, cef=ap.cef, eig=ap.eig}
      mask prompts: ceb "Control effectiveness body struct"; cef "Control effectiveness flaps struct"; eig "Eigendynamics struct"
  INDI control allocation : ca_lib/INDI wls control allocation  ca=ap.ca  is_Delta_u_d_checked=on  is_Delta_gamma_checked=off  is_Delta_W_v_checked=off  is_Delta_u_max_checked=off  is_W_checked=off  is_iter_checked=on
      settings: SourceProductName=LADAC
  Mux : Mux  Inputs=2
  Mux1 : Mux  Inputs=2
  Only rotational control effectiveness : MATLAB Function  TreatAsAtomicUnit=on
  Saturation2 : Saturate  UpperLimit=ap.ca.u_max  LowerLimit=ap.ca.u_min
  Saturation3 : Saturate  UpperLimit=ap.ca.u_max  LowerLimit=ap.ca.u_min
  Sensor Filter : filters_lib/T2 Filter (Discrete)  omega_0=ap.sflt.omega  d=ap.sflt.d  Ts=ap_notune.ts  is_vel=false  is_acc=false  SimulateUsing=Code generation
      settings: SourceProductName=LADAC
  Servo Dynamics : filters_lib/PT2 discrete with saturation  param_src=internal  omega=ap.servo.omega  d=ap.servo.d  x_max=inf  x_min=-inf  x_dt_max=inf  x_dt_min=-inf  x_dt2_max=inf  x_dt2_min=-inf  y_0_src=internal  x_init=0  y_dt_0_src=internal  x_dt_init=0  is_y_dt_checked=off  is_y_dt2_checked=off  is_external_reset_checked=off  mask_expr_handling_config=default
      settings: SourceProductName=LADAC
  Servo delay : Subsystem
  T2 servo booster : Subsystem  mask{omega=ap.servo.omega, d=ap.servo.d, b=ap.servo.boost}
      mask prompts: omega "Eigenfrequency, rad/s"; d "Damping Ratio"; b "Booster Factor"
      mask DialogControl DescGroupVar Prompt: T2 Booster
  T2 servo booster1 : $bdroot/LindiPlane Autopilot/Plane Inner Loop INDI and Control Allocation/T2 servo booster  omega=ap.servo.omega  d=ap.servo.d  b=ap.servo.boost
  Uaero booster : Subsystem  mask{uaero_use=ap.uaero.use, opt1=ap.uaero.opt1, opt2=ap.uaero.opt2, Vref=ap.uaero.Vref, uaero=ap.uaero, A1=0.165, b1=0.0455, A2=0.335, b2=0.3}
      mask prompts: uaero_use "Enable"; opt1 "Option 1"; opt2 "Option 2"; uaero "Unsteady aerodynamics struct"
      mask DialogControl DescGroupVar Prompt: T2 Booster
  Uaero booster1 : $bdroot/LindiPlane Autopilot/Plane Inner Loop INDI and Control Allocation/Uaero booster  uaero_use=ap.uaero.use  opt1=ap.uaero.opt1  opt2=ap.uaero.opt2  Vref=ap.uaero.Vref  uaero=ap.uaero  A1=0.165  b1=0.0455  A2=0.335  b2=0.3
  Unit Delay : UnitDelay  SampleTime=-1  HasFrameUpgradeWarning=on
  Unsteady aerodynamics : Subsystem  mask{uaero_use=ap.uaero.use}
      mask prompts: uaero_use "Enable"
  control effectiveness : Subsystem  mask{ceb=ap.ceb, cef=ap.cef, eig=ap.eig}
      mask prompts: ceb "Rigid-body control effectiveness struct"; cef "Flaps control effectiveness struct"; eig "State dynamics struct"
  inner_loop_indi : Outport  VectorParamsAs1DForOutWhenUnconnected=off
  wires:
  Avoid Chattering/1(Delta_u_last) -> Add3/2
  control effectiveness/2(Gdw) -> Flap downwash compensation/1(Gdw), Direct lift control - control allocation/3(Gdw), Add5/2
  control effectiveness/1(G1) -> Add5/1  "G1"
  Delta u_d/1(Delta_u) -> Add3/1
  Add3/1 -> Flap downwash compensation/3(Delta_u)
  Uaero booster1/1 -> Add4/1
  T2 servo booster1/1 -> Uaero booster1/1
  Add2/1 -> INDI control allocation/3, Avoid Chattering/1(u)
  Unit Delay/1 -> Add/1
  De-activate DLC at high pitch angle errors/1(Delta_nu_acc_z_out) -> Add/2
  Compare To Constant1/1 -> Collective ailerons decay/Enable, De-activate DLC at high pitch angle errors/Enable
  Add/1 -> Mux1/2
  Uaero booster/1(u_boost) -> Saturation3/1
  V_A/1 -> control effectiveness/1(V), Flap downwash compensation/2(V), Direct lift control - control allocation/6(V), Uaero booster/2(V_A), Uaero booster1/2, Unsteady aerodynamics/2(V)
  Unsteady aerodynamics/1(u_unst) -> Sensor Filter/1, Add2/2
  Direct lift control - control allocation/1(u) -> Add4/3
  e_Theta/1 -> Direct lift control - control allocation/5(e_Theta), De-activate DLC at high pitch angle errors/2(e_Theta)
  Delta_nu_acc_z/1 -> Direct lift control - control allocation/4(Delta_nu_acc_z), De-activate DLC at high pitch angle errors/1(Delta_nu_acc_z)
  Collective ailerons decay/1(Delta nu_acc_z) -> Unit Delay/1
  Constant/1 -> Compare To Constant/1, Only rotational control effectiveness/2(DLC_opt), Compare To Constant1/1
  Compare To Constant/1 -> Direct lift control - control allocation/Enable
  Saturation2/1 -> Mux/1  "u"
  Add4/1 -> Saturation2/1
  T2 servo booster/1(u_boost) -> Uaero booster/1(u)
  Servo Dynamics/1 -> Bus Creator/4, Unsteady aerodynamics/1(u)  "u_bar"
  Servo delay/1(u_delay) -> Servo Dynamics/1
  Flap downwash compensation/1(Delta_nu_dw) -> Add1/2
  Add1/1 -> INDI control allocation/2
  Delta_nu_Omega_Kb_dt/1 -> Mux1/1
  INDI control allocation/2 -> Bus Creator/7  "iter"
  rho/1 -> control effectiveness/2(rho)
  Mux/1 -> Bus Creator/3  "u"
  throttle_0_1/1 -> Mux/2
  Mux1/1 -> Add1/1, Bus Creator/6  "Delta_nu"
  Add5/1 -> Bus Creator/1, Only rotational control effectiveness/1(G)  "G1"
  Bus Creator/1 -> inner_loop_indi/1
  Add6/1 -> T2 servo booster/1(u), Direct lift control - control allocation/1(u_in)
  Sensor Filter/1 -> Add6/2, Bus Creator/5  "u_bar_f"
  Saturation3/1 -> Servo delay/1(u), Add4/2, Collective ailerons decay/2(u)  "u"
  Only rotational control effectiveness/1(G4xX) -> Direct lift control - control allocation/2(G1), INDI control allocation/1  "G1"
  INDI control allocation/1 -> Bus Creator/2, Add6/1, Avoid Chattering/2(Delta_u)  "Delta_u"
  u_d/1 -> Collective ailerons decay/1(Delta u_d), Delta u_d/1(u), Add2/1, INDI control allocation/4, T2 servo booster1/1

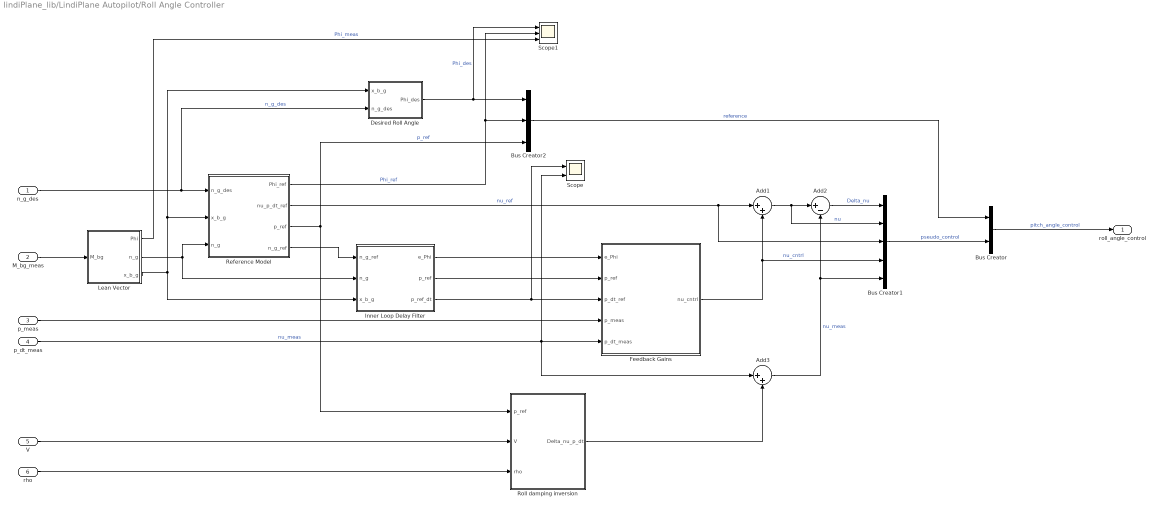
== system lindiPlane_lib/LindiPlane Autopilot/Roll Angle Controller ==
  n_g_des : Inport
  M_bg_meas : Inport  Port=2
  p_meas : Inport  Port=3
  p_dt_meas : Inport  Port=4
  V : Inport  Port=5
  rho : Inport  Port=6
  Add1 : Sum  Inputs=|++
  Add2 : Sum  Inputs=|+-
  Add3 : Sum  Inputs=|++
  Bus Creator : BusCreator  Inputs=2
  Bus Creator1 : BusCreator  Inputs=5
  Bus Creator2 : BusCreator  Inputs=3
  Desired Roll Angle : MATLAB Function  TreatAsAtomicUnit=on
  Feedback Gains : Subsystem
  Inner Loop Delay Filter : Subsystem
  Lean Vector : Subsystem
  Reference Model : Subsystem
  Roll damping inversion : Subsystem
  Scope : Scope  NumInputPorts=2
  Scope1 : Scope  NumInputPorts=3
  roll_angle_control : Outport  VectorParamsAs1DForOutWhenUnconnected=off
  wires:
  Reference Model/1(Phi_ref) -> Bus Creator2/2, Scope1/2  "Phi_ref"
  Lean Vector/1(Phi) -> Scope1/3  "Phi_meas"
  Inner Loop Delay Filter/3(p_ref_dt) -> Feedback Gains/3(p_dt_ref), Scope/1
  Inner Loop Delay Filter/2(p_ref) -> Feedback Gains/2(p_ref)
  Inner Loop Delay Filter/1(e_Phi) -> Feedback Gains/1(e_Phi)
  Reference Model/4(n_g_ref) -> Inner Loop Delay Filter/1(n_g_ref)
  Reference Model/3(p_ref) -> Bus Creator2/3, Roll damping inversion/1(p_ref)  "p_ref"
  Reference Model/2(nu_p_dt_ref) -> Add1/1, Bus Creator1/3  "nu_ref"
  Desired Roll Angle/1(Phi_des) -> Bus Creator2/1, Scope1/1  "Phi_des"
  Lean Vector/3(x_b_g) -> Inner Loop Delay Filter/3(x_b_g), Reference Model/2(x_b_g), Desired Roll Angle/1(x_b_g)
  Lean Vector/2(n_g) -> Inner Loop Delay Filter/2(n_g), Reference Model/3(n_g)
  M_bg_meas/1 -> Lean Vector/1(M_bg)
  n_g_des/1 -> Reference Model/1(n_g_des), Desired Roll Angle/2(n_g_des)  "n_g_des"
  Roll damping inversion/1(Delta_nu_p_dt) -> Add3/2
  Add3/1 -> Bus Creator1/5, Add2/2  "nu_meas"
  rho/1 -> Roll damping inversion/3(rho)
  V/1 -> Roll damping inversion/2(V)
  Add1/1 -> Add2/1, Bus Creator1/2  "nu"
  Bus Creator1/1 -> Bus Creator/2  "pseudo_control"
  Bus Creator/1 -> roll_angle_control/1  "pitch_angle_control"
  Add2/1 -> Bus Creator1/1  "Delta_nu"
  p_dt_meas/1 -> Scope/2, Add3/1, Feedback Gains/5(p_dt_meas)  "nu_meas"
  Feedback Gains/1(nu_cntrl) -> Add1/2, Bus Creator1/4  "nu_cntrl"
  p_meas/1 -> Feedback Gains/4(p_meas)
  Bus Creator2/1 -> Bus Creator/1  "reference"

== system lindiPlane_lib/LindiPlane Autopilot/Rudder Decay Controller ==
  u : Inport
  Gain5 : Gain  Gain=ap.atc.rm.ydecaytc
  Rudder command : MATLAB Function  TreatAsAtomicUnit=on
  Unit Delay : UnitDelay  SampleTime=-1  HasFrameUpgradeWarning=on
  r_cmd : Outport  VectorParamsAs1DForOutWhenUnconnected=off
  wires:
  Unit Delay/1 -> r_cmd/1
  u/1 -> Rudder command/1(u)
  Rudder command/1(y) -> Gain5/1
  Gain5/1 -> Unit Delay/1

== system lindiPlane_lib/LindiPlane Autopilot/Sstick Command Bus ==
  cmd_roll : Inport
  cmd_pitch : Inport  Port=2
  cmd_yaw : Inport  Port=3
  cmd_throttle : Inport  Port=4
  Bus Creator : BusCreator  Inputs=4
  stickCmdBus : Outport  VectorParamsAs1DForOutWhenUnconnected=off
  wires:
  cmd_throttle/1 -> Bus Creator/4  "cmd_throttle"
  cmd_yaw/1 -> Bus Creator/3  "cmd_yaw"
  cmd_pitch/1 -> Bus Creator/2  "cmd_pitch"
  Bus Creator/1 -> stickCmdBus/1
  cmd_roll/1 -> Bus Creator/1  "cmd_roll"

== system lindiPlane_lib/LindiPlane Autopilot/Turn Coordination ==
  Phi_ref_ff : Inport
  r_cmd_in : Inport  Port=2
  V : Inport  Port=3
  Enable : EnablePort
  Add : Sum
  Turn Coordination : MATLAB Function  TreatAsAtomicUnit=on
  q_cmd : Outport  VectorParamsAs1DForOutWhenUnconnected=off
  r_cmd : Outport  Port=2  VectorParamsAs1DForOutWhenUnconnected=off
  wires:
  r_cmd_in/1 -> Add/2
  Add/1 -> r_cmd/1
  Turn Coordination/2(r) -> Add/1
  V/1 -> Turn Coordination/2(V)
  Phi_ref_ff/1 -> Turn Coordination/1(Phi)
  Turn Coordination/1(q) -> q_cmd/1

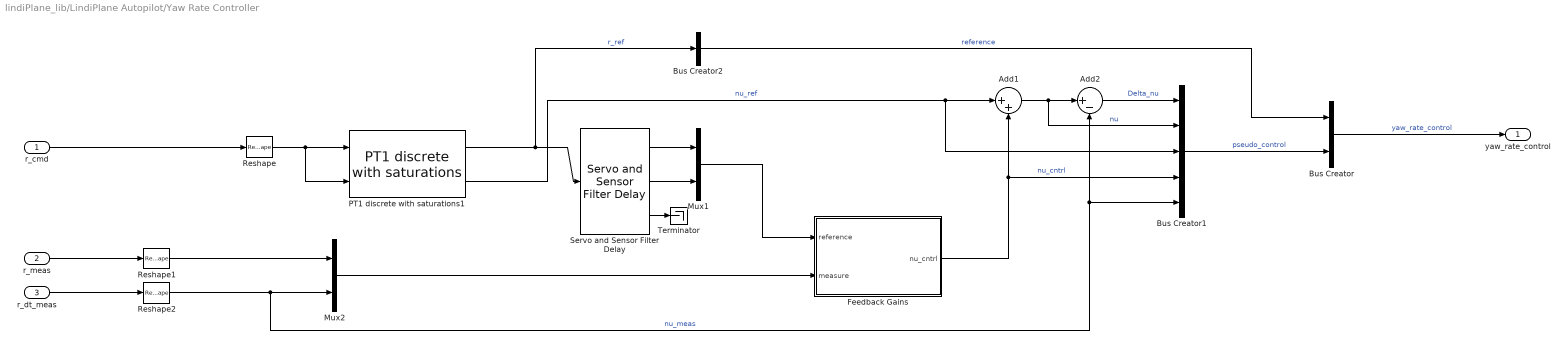
== system lindiPlane_lib/LindiPlane Autopilot/Yaw Rate Controller ==
  r_cmd : Inport
  r_meas : Inport  Port=2
  r_dt_meas : Inport  Port=3
  Add1 : Sum  Inputs=|++
  Add2 : Sum  Inputs=|+-
  Bus Creator : BusCreator  Inputs=2
  Bus Creator1 : BusCreator  Inputs=5
  Bus Creator2 : BusCreator  Inputs=1
  Feedback Gains : Subsystem
  Mux1 : Mux  Inputs=2
  Mux2 : Mux  Inputs=2
  PT1 discrete with saturations1 : filters_lib/PT1 discrete with saturations  param_src=internal  T=1/ap.atc.rm.yfreq  x_max=inf  x_min=-inf  x_dt_max=inf  x_dt_min=-inf  y_0_src=external  x_init=0  is_y_dt_checked=on  is_external_reset_checked=off  mask_expr_handling_config=passthrough (tunable)
      settings: SourceProductName=LADAC
  Reshape : Reshape
  Reshape1 : Reshape
  Reshape2 : Reshape
  Servo and Sensor Filter Delay : $bdroot/LindiPlane Autopilot/Pitch Angle Controller/Servo and Sensor Filter Delay  SystemSampleTime=-1  VariantActivationTime=update diagram  AllowFlexibleInterface=on  Latency=0  AutoFrameSizeCalculation=off
  Terminator : Terminator
  yaw_rate_control : Outport  VectorParamsAs1DForOutWhenUnconnected=off
  wires:
  Reshape2/1 -> Bus Creator1/5, Add2/2, Mux2/2  "nu_meas"
  Reshape1/1 -> Mux2/1
  Servo and Sensor Filter Delay/3 -> Terminator/1
  Servo and Sensor Filter Delay/1 -> Mux1/1
  Servo and Sensor Filter Delay/2 -> Mux1/2
  Feedback Gains/1(nu_cntrl) -> Bus Creator1/4, Add1/2  "nu_cntrl"
  Add2/1 -> Bus Creator1/1  "Delta_nu"
  Mux2/1 -> Feedback Gains/2(measure)
  r_cmd/1 -> Reshape/1
  PT1 discrete with saturations1/2 -> Bus Creator1/3, Add1/1  "nu_ref"
  Bus Creator2/1 -> Bus Creator/1  "reference"
  r_dt_meas/1 -> Reshape2/1
  Bus Creator/1 -> yaw_rate_control/1  "yaw_rate_control"
  PT1 discrete with saturations1/1 -> Bus Creator2/1, Servo and Sensor Filter Delay/1  "r_ref"
  Add1/1 -> Add2/1, Bus Creator1/2  "nu"
  r_meas/1 -> Reshape1/1
  Bus Creator1/1 -> Bus Creator/2  "pseudo_control"
  Mux1/1 -> Feedback Gains/1(reference)
  Reshape/1 -> PT1 discrete with saturations1/1, PT1 discrete with saturations1/2

== system lindiPlane_lib/LindiPlane Autopilot/add ==
  In1 : Inport
  In2 : Inport  Port=2
  Enable : EnablePort
  Add2 : Sum
  Out1 : Outport  VectorParamsAs1DForOutWhenUnconnected=off
  wires:
  In2/1 -> Add2/2
  In1/1 -> Add2/1
  Add2/1 -> Out1/1

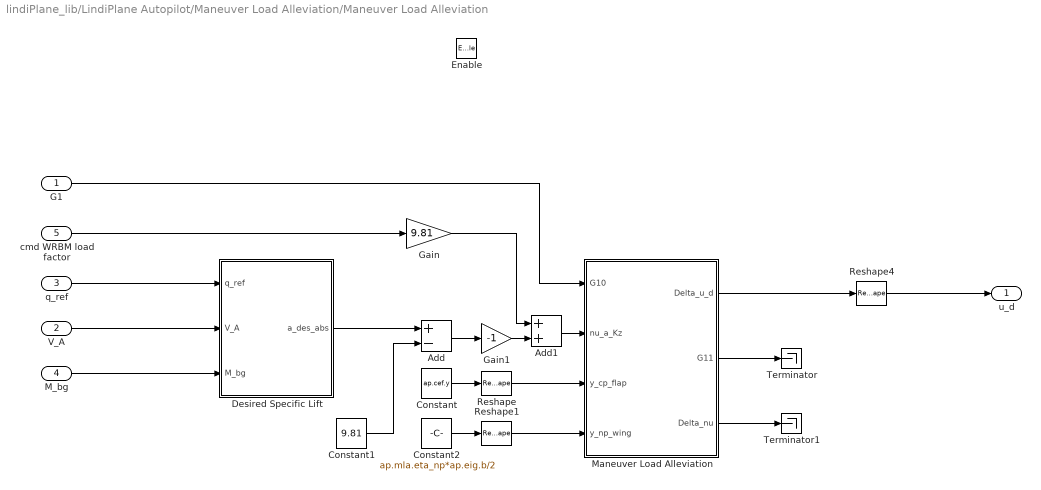
== system lindiPlane_lib/LindiPlane Autopilot/Maneuver Load Alleviation/Maneuver Load Alleviation ==
  G1 : Inport
  V_A : Inport  Port=2
  q_ref : Inport  Port=3
  M_bg : Inport  Port=4
  cmd WRBM load factor : Inport  Port=5
  Enable : EnablePort  StatesWhenEnabling=reset
  Add : Sum  Inputs=+-
  Add1 : Sum
  Constant : Constant  Value=ap.cef.y
  Constant1 : Constant  Value=9.81
  Constant2 : Constant  Value=ap.mla.eta_np*ap.eig.b/2
  Desired Specific Lift : Subsystem
  Gain : Gain  Gain=9.81
  Gain1 : Gain  Gain=-1
  Maneuver Load Alleviation : MATLAB Function  TreatAsAtomicUnit=on
  Reshape : Reshape  OutputDimensionality=Row vector (2-D)
  Reshape1 : Reshape  OutputDimensionality=Row vector (2-D)
  Reshape4 : Reshape
  Terminator : Terminator
  Terminator1 : Terminator
  u_d : Outport  VectorParamsAs1DForOutWhenUnconnected=off
  wires:
  Add1/1 -> Maneuver Load Alleviation/2(nu_a_Kz)
  Gain/1 -> Add1/1
  cmd WRBM load factor/1 -> Gain/1
  Maneuver Load Alleviation/3(Delta_nu) -> Terminator1/1
  Maneuver Load Alleviation/2(G11) -> Terminator/1
  q_ref/1 -> Desired Specific Lift/1(q_ref)
  Constant2/1 -> Reshape1/1
  V_A/1 -> Desired Specific Lift/2(V_A)
  G1/1 -> Maneuver Load Alleviation/1(G10)
  Reshape4/1 -> u_d/1
  Constant/1 -> Reshape/1
  Constant1/1 -> Add/2
  Add/1 -> Gain1/1
  Gain1/1 -> Add1/2
  Reshape1/1 -> Maneuver Load Alleviation/4(y_np_wing)
  Maneuver Load Alleviation/1(Delta_u_d) -> Reshape4/1
  Reshape/1 -> Maneuver Load Alleviation/3(y_cp_flap)
  Desired Specific Lift/1(a_des_abs) -> Add/1
  M_bg/1 -> Desired Specific Lift/3(M_bg)

== system lindiPlane_lib/LindiPlane Autopilot/Maneuver Load Alleviation/Subsystem ==
  Enable : EnablePort
  Constant : Constant  Value=ap.ca.u_d
  u_d : Outport  VectorParamsAs1DForOutWhenUnconnected=off
  wires:
  Constant/1 -> u_d/1

== system lindiPlane_lib/LindiPlane Autopilot/Measurement Filtering/Acc Filter ==
  a_Kb : Inport
  Compare To Constant1 : simulink/Logic and Bit Operations/Compare To Constant  relop=>  const=2  OutDataTypeStr=boolean
  Constant2 : Constant  Value=ap.dlc.opt
  Logical Operator1 : Logic  Operator=NOT  AllPortsSameDT=off  OutDataTypeStr=boolean
  Merge2 : Merge
  Reshape : Reshape
  Subsystem : Subsystem
  Subsystem1 : Subsystem
  a_Kb_F : Outport  VectorParamsAs1DForOutWhenUnconnected=off
  wires:
  Reshape/1 -> a_Kb_F/1
  Merge2/1 -> Reshape/1
  a_Kb/1 -> Subsystem/1(a_Kb), Subsystem1/1(a_Kb)
  Subsystem1/1(a_Kb_F) -> Merge2/2
  Compare To Constant1/1 -> Subsystem/Enable, Logical Operator1/1
  Subsystem/1(a_Kb_F) -> Merge2/1
  Logical Operator1/1 -> Subsystem1/Enable
  Constant2/1 -> Compare To Constant1/1

== system lindiPlane_lib/LindiPlane Autopilot/Measurement Filtering/Duplicate LPF ==
  Omega_Kb : Inport
  Enable : EnablePort
  T2 Filter (Discrete)1 : filters_lib/T2 Filter (Discrete)  omega_0=2*ap.sflt.omega  d=sqrt(ap.sflt.d)  Ts=ap_notune.ts  is_vel=true  is_acc=false  SimulateUsing=Code generation
      settings: SourceProductName=LADAC
  T2 Filter (Discrete)3 : filters_lib/T2 Filter (Discrete)  omega_0=2*ap.sflt.omega  d=sqrt(ap.sflt.d)  Ts=ap_notune.ts  is_vel=false  is_acc=false  SimulateUsing=Code generation
      settings: SourceProductName=LADAC
  Omega_Kb_f : Outport  VectorParamsAs1DForOutWhenUnconnected=off
  Omega_Kb_dt_f : Outport  Port=2  VectorParamsAs1DForOutWhenUnconnected=off
  wires:
  T2 Filter (Discrete)3/1 -> T2 Filter (Discrete)1/1  "M_bg_f"
  Omega_Kb/1 -> T2 Filter (Discrete)3/1
  T2 Filter (Discrete)1/2 -> Omega_Kb_dt_f/1
  T2 Filter (Discrete)1/1 -> Omega_Kb_f/1

== system lindiPlane_lib/LindiPlane Autopilot/Measurement Filtering/Single LPF ==
  Omega_Kb : Inport
  Enable : EnablePort
  T2 Filter (Discrete)3 : filters_lib/T2 Filter (Discrete)  omega_0=ap.sflt.omega  d=ap.sflt.d  Ts=ap_notune.ts  is_vel=true  is_acc=false  SimulateUsing=Code generation
      settings: SourceProductName=LADAC
  Omega_Kb_f : Outport  VectorParamsAs1DForOutWhenUnconnected=off
  Omega_Kb_dt_f : Outport  Port=2  VectorParamsAs1DForOutWhenUnconnected=off
  wires:
  Omega_Kb/1 -> T2 Filter (Discrete)3/1
  T2 Filter (Discrete)3/2 -> Omega_Kb_dt_f/1
  T2 Filter (Discrete)3/1 -> Omega_Kb_f/1

== system lindiPlane_lib/LindiPlane Autopilot/Pitch Angle Controller/Servo and Sensor Filter Delay ==
  ref : Inport
  PT2 discrete with saturation5 : filters_lib/PT2 discrete with saturation  param_src=internal  omega=ap.servo.omega*ap.servo.boost  d=ap.servo.d  x_max=inf  x_min=-inf  x_dt_max=inf  x_dt_min=-inf  x_dt2_max=inf  x_dt2_min=-inf  y_0_src=external  x_init=0  y_dt_0_src=internal  x_dt_init=0  is_y_dt_checked=off  is_y_dt2_checked=off  is_external_reset_checked=off  mask_expr_handling_config=passthrough (tunable)
      settings: SourceProductName=LADAC
  Reshape : Reshape
  Reshape1 : Reshape
  Reshape2 : Reshape
  Sensor Filter : filters_lib/T2 Filter (Discrete)  omega_0=ap.sflt.omega  d=ap.sflt.d  Ts=ap_notune.ts  is_vel=true  is_acc=true  SimulateUsing=Code generation
      settings: SourceProductName=LADAC
  Servo delay : $bdroot/LindiPlane Autopilot/Plane Inner Loop INDI and Control Allocation/Servo delay  SystemSampleTime=-1  VariantActivationTime=update diagram  AllowFlexibleInterface=on  Latency=0  AutoFrameSizeCalculation=off
  Unsteady Aerodynamics : Subsystem
  ref_f : Outport  VectorParamsAs1DForOutWhenUnconnected=off
  ref_dt_f : Outport  Port=2  VectorParamsAs1DForOutWhenUnconnected=off
  ref_dt2_f : Outport  Port=3  VectorParamsAs1DForOutWhenUnconnected=off
  wires:
  ref/1 -> Servo delay/1, PT2 discrete with saturation5/2
  Sensor Filter/1 -> Reshape/1
  Sensor Filter/2 -> Reshape1/1
  Sensor Filter/3 -> Reshape2/1
  PT2 discrete with saturation5/1 -> Unsteady Aerodynamics/1(u)
  Servo delay/1 -> PT2 discrete with saturation5/1
  Unsteady Aerodynamics/1(u_unst) -> Sensor Filter/1
  Reshape/1 -> ref_f/1
  Reshape1/1 -> ref_dt_f/1
  Reshape2/1 -> ref_dt2_f/1

== system lindiPlane_lib/LindiPlane Autopilot/Pitch Rate Controller/Feedback Gains ==
  reference : Inport
  measure : Inport  Port=2
  Add : Sum  Inputs=2
  Add1 : Sum  Inputs=|+-
  Add2 : Sum  Inputs=|+-
  Demux : Demux  Outputs=2
  Demux1 : Demux  Outputs=2
  Gain3 : Gain  Gain=ap.atc.k.prat
  Gain5 : Gain  Gain=ap.atc.k.pacc
  nu_cntrl : Outport  VectorParamsAs1DForOutWhenUnconnected=off
  wires:
  Add/1 -> nu_cntrl/1
  Gain3/1 -> Add/1
  Gain5/1 -> Add/2
  Demux/2 -> Add2/1
  Demux/1 -> Add1/1
  reference/1 -> Demux/1
  measure/1 -> Demux1/1
  Add1/1 -> Gain3/1
  Add2/1 -> Gain5/1
  Demux1/1 -> Add1/2
  Demux1/2 -> Add2/2

== system lindiPlane_lib/LindiPlane Autopilot/Pitch Rate Controller/Pitch eigendynamics ==
  q_ref : Inport
  V : Inport  Port=2
  rho : Inport  Port=3
  Add2 : Sum  Inputs=|+-
  Add5 : Sum
  Gain8 : Gain  Gain=1/ap.ceb.iyy
  Pitch damping : Subsystem
  Pitch stiffness : Subsystem
  Servo and Sensor Filter Delay : $bdroot/LindiPlane Autopilot/Pitch Angle Controller/Servo and Sensor Filter Delay  SystemSampleTime=-1  VariantActivationTime=update diagram  AllowFlexibleInterface=on  Latency=0  AutoFrameSizeCalculation=off
  Terminator : Terminator
  Terminator1 : Terminator
  Delta_nu_q_dt : Outport  VectorParamsAs1DForOutWhenUnconnected=off
  wires:
  Servo and Sensor Filter Delay/3 -> Terminator1/1
  Servo and Sensor Filter Delay/2 -> Terminator/1
  Servo and Sensor Filter Delay/1 -> Add2/2
  Pitch stiffness/1(Delta_M) -> Add5/2
  Pitch damping/1(Delta_M) -> Add5/1
  Add2/1 -> Pitch stiffness/1(Delta_q_ref), Pitch damping/1(Delta_q_ref)
  Add5/1 -> Gain8/1
  rho/1 -> Pitch damping/3(rho), Pitch stiffness/3(rho)
  q_ref/1 -> Add2/1, Servo and Sensor Filter Delay/1
  V/1 -> Pitch stiffness/2(V), Pitch damping/2(V)
  Gain8/1 -> Delta_nu_q_dt/1
